simulink library "PAC_online_tuning_blocks"  (R2025a)
settings: Solver=VariableStepAuto  StartTime=0.0  StopTime=10.0  RelTol=1e-3
settings Model: Creator=dperera  LastModifiedBy=dperera

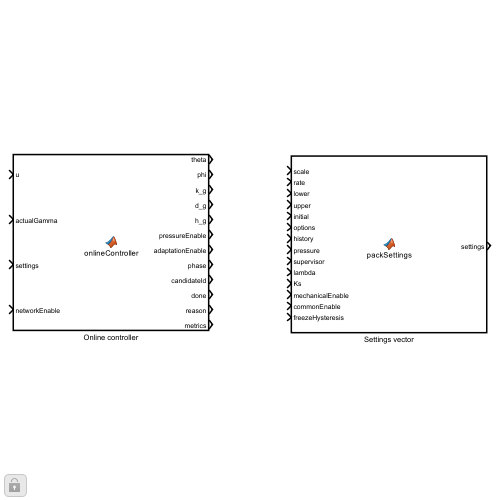
[thumbnail: Simulink's stored preview of the top-level diagram]
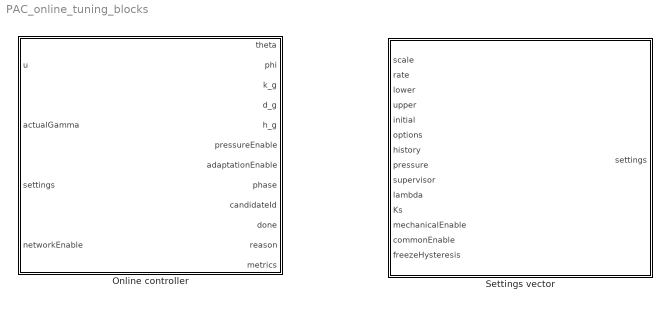
== system PAC_online_tuning_blocks ==
  Online controller : MATLAB Function  TreatAsAtomicUnit=on
  Settings vector : MATLAB Function  TreatAsAtomicUnit=on

== matlab function PAC_online_tuning_blocks/Settings vector ==
  data: scale input size=[10 1]; settings output size=[81 1]; rate input size=[10 1]; lower input size=[10 1]; upper input size=[10 1]; initial input size=[10 1]; options input size=[3 1]; history input size=[4 1]; pressure input size=[10 1]; supervisor input size=[7 1]; lambda input size=[2 1]; Ks input size=[2 1]; mechanicalEnable input; commonEnable input; freezeHysteresis input
function settings = packSettings(scale,rate,lower,upper,initial,options,history,pressure,supervisor,lambda,Ks,mechanicalEnable,commonEnable,freezeHysteresis)
%#codegen
settings=pacOnlineSettingsVector(scale,rate,lower,upper,initial,options,history,pressure,supervisor,lambda,Ks,mechanicalEnable,commonEnable,freezeHysteresis);
end

== matlab function PAC_online_tuning_blocks/Online controller ==
  settings: updateMethod=DISCRETE  sampleTime=0.05
  data: u input size=[12 1]; theta output; actualGamma input size=[10 1]; settings input size=[81 1]; networkEnable input; phi output; k_g output; d_g output; h_g output; pressureEnable output; adaptationEnable output; phase output; candidateId output; done output; reason output; metrics output size=[4 1]
function [theta,phi,k_g,d_g,h_g,pressureEnable,adaptationEnable,phase,candidateId,done,reason,metrics] = onlineController(u,actualGamma,settings,networkEnable)
%#codegen
coder.extrinsic('pacOnlineUdpBridge');
data=coder.load('C:\Users\dperera\OneDrive - Texas A&M University\Lab\Research\fDyn_ExpCom\hyDyn_Ctrl\passivity_adaptive_control\autotuning\online_sessions\phi1_T5_scale5_initial\pacOnlineSession.mat','rt'); c=data.rt;
persistent state
if isempty(state),state=pacOnlineInitialState(c);end
rx=zeros(7,1);
% Transmit the complete previous sample, keeping all timestamps aligned.
persistent packet
if isempty(packet),packet=zeros(121,1);packet(1)=c.session;packet(5)=-1;end
if networkEnable,rx=pacOnlineUdpBridge(packet,c.blockPort,c.workerPort,c.session);end
[state,y,header]=pacOnlineRuntimeStep(state,u,actualGamma,settings,rx,c);
packet=[header;u;y(1:2);actualGamma;settings];
theta=y(1);phi=y(2);k_g=y(3);d_g=y(4);h_g=y(5);
pressureEnable=y(6);adaptationEnable=y(7);
phase=y(8);candidateId=y(9);done=y(10);reason=y(11);metrics=y(12:15);
end
